simulink model "battery"  (R2026a)
settings: Solver=VariableStepAuto
undefined symbols (not defined in the file or in its folder): batt
settings Model: Creator=flow  LastModifiedBy=flow

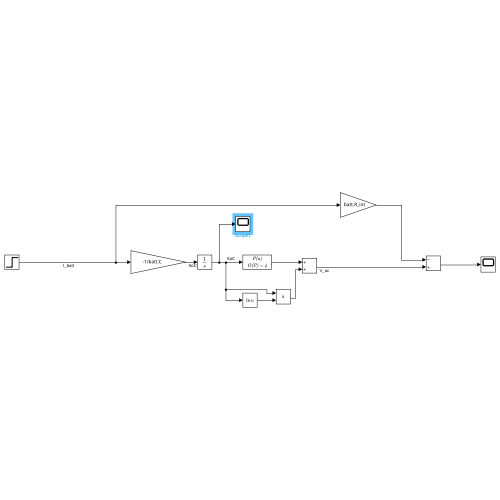
[thumbnail: Simulink's stored preview of the top-level diagram]
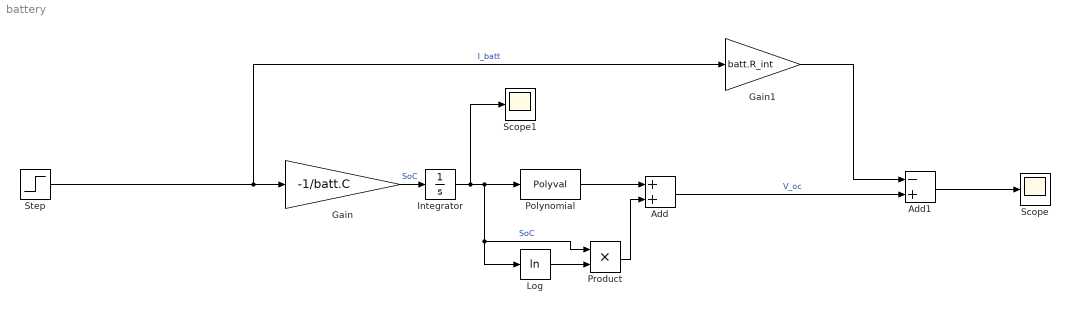
== system battery ==
  Add : Sum
  Add1 : Sum  Inputs=-+
  Gain : Gain  Gain=-1/batt.C
  Gain1 : Gain  Gain=batt.R_int
  Integrator : Integrator  InitialCondition=1
  Log : Math  Operator=log
  Polynomial : Polyval  Coefs=batt.Pol_ocv
  Product : Product
  Scope : Scope
      settings: ActiveDisplayYMinimum=10.090020291236856  ActiveDisplayYMaximum=10.695465879390186
  Scope1 : Scope
      settings: ActiveDisplayYMinimum=0.99350961538461657  ActiveDisplayYMaximum=1.0007211538461538
  Step : Step  FinalValue=3  SampleTime=0
  wires:
  Integrator/1 -> Scope1/1, Log/1, Product/1, Polynomial/1  "SoC"
  Step/1 -> Gain1/1, Gain/1  "I_batt"
  Polynomial/1 -> Add/1
  Log/1 -> Product/2
  Product/1 -> Add/2
  Add/1 -> Add1/2  "V_oc"
  Gain1/1 -> Add1/1
  Add1/1 -> Scope/1
  Gain/1 -> Integrator/1  "SoC"
